simulink model "quad_closed_loop"  (R2024a)
settings: Solver=ode4  StartTime=0.0  StopTime=14  FixedStep=1e-3  RelTol=1e-3
settings Model: Creator=qixiaoyang  LastModifiedBy=qixiaoyang

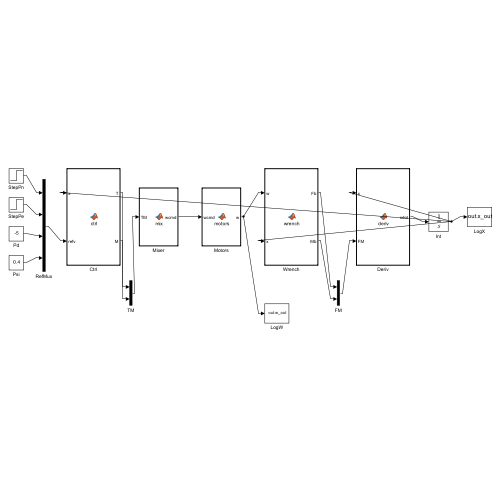
[thumbnail: Simulink's stored preview of the top-level diagram]
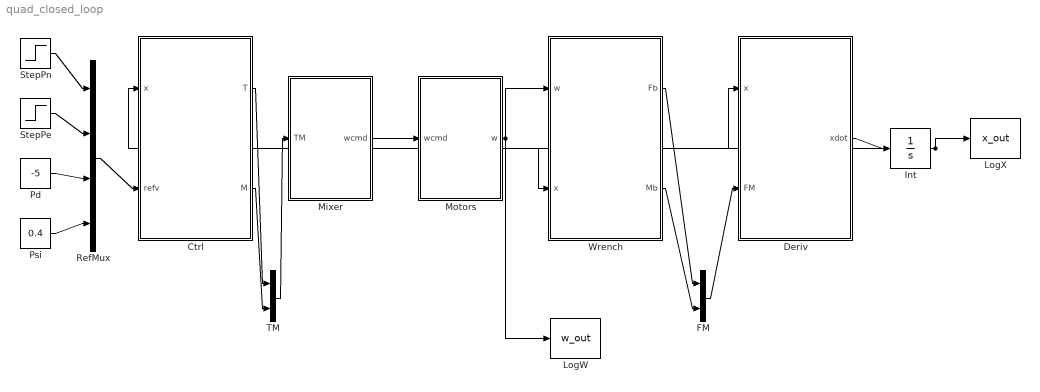
== system quad_closed_loop ==
  Ctrl : MATLAB Function  TreatAsAtomicUnit=on
  Deriv : MATLAB Function  TreatAsAtomicUnit=on
  FM : Mux  Inputs=2
  Int : Integrator  InitialCondition=[0;0;-5;0;0;0;1;0;0;0;0;0;0]
  LogW : ToWorkspace  VariableName=w_out  SaveFormat=Timeseries  SampleTime=-1
  LogX : ToWorkspace  VariableName=x_out  SaveFormat=Timeseries  SampleTime=-1
  Mixer : MATLAB Function  TreatAsAtomicUnit=on
  Motors : MATLAB Function  TreatAsAtomicUnit=on
  Pd : Constant  Value=-5
  Psi : Constant  Value=0.4
  RefMux : Mux
  StepPe : Step  After=2  SampleTime=0
  StepPn : Step  After=3  SampleTime=0
  TM : Mux  Inputs=2
  Wrench : MATLAB Function  TreatAsAtomicUnit=on
  wires:
  StepPn/1 -> RefMux/1
  StepPe/1 -> RefMux/2
  Pd/1 -> RefMux/3
  Psi/1 -> RefMux/4
  Int/1 -> Ctrl/1(x), Wrench/2(x), Deriv/1(x), LogX/1
  RefMux/1 -> Ctrl/2(refv)
  Ctrl/1(T) -> TM/1
  Ctrl/2(M) -> TM/2
  TM/1 -> Mixer/1(TM)
  Mixer/1(wcmd) -> Motors/1(wcmd)
  Motors/1(w) -> Wrench/1(w), LogW/1
  Wrench/1(Fb) -> FM/1
  Wrench/2(Mb) -> FM/2
  FM/1 -> Deriv/2(FM)
  Deriv/1(xdot) -> Int/1

== matlab function quad_closed_loop/Ctrl ==
  settings: updateMethod=DISCRETE  sampleTime=1e-3
  data: x input; T output; refv input; M output
function [T, M] = ctrl(x, refv)
% 级联控制器：位置环 -> 推力方向 -> 姿态环
persistent st
if isempty(st)
    st.ip = [0;0;0];
    st.ia = [0;0;0];
end
pn = x(1:3); Vb = x(4:6); q = x(7:10); w = x(11:13);
R = dcm(q);
Vn = R*Vb;
ep = refv(1:3) - pn;
ev = -Vn;
a = [1.6000000000000001;1.6000000000000001;2.5].*ep + [2.2000000000000002;2.2000000000000002;3].*ev + [0;0;1.2].*st.ip;
aHor = a(1:2);
aMax = 9.8100000000000005*tan(0.6108652381980153);
if norm(aHor) > aMax
    a(1:2) = aHor*(aMax/norm(aHor));
end
st.ip = st.ip + ep*0.001;
st.ip = min(max(st.ip, -[0;0;1]), [0;0;1]);
v = [0;0;9.8100000000000005] - a;
nv = norm(v);
if nv < 1e-6
    v = [0;0;1]; nv = 1;
end
z = v/nv;
T = 1.5*nv;
T = min(max(T, 0), 40);
psi = refv(4);
xc = [cos(psi); sin(psi); 0];
yb = cross(z, xc);
ny = norm(yb);
if ny < 1e-6
    xc = [1;0;0]; yb = cross(z, xc); ny = norm(yb);
end
yb = yb/ny;
xb = cross(yb, z);
Rd = [xb yb z];
phiD = atan2(Rd(3,2), Rd(3,3));
thetaD = -asin(max(-1, min(1, Rd(3,1))));
psiD = atan2(Rd(2,1), Rd(1,1));
att = euler(q);
e = [phiD;thetaD;psiD] - att;
e = mod(e + pi, 2*pi) - pi;
st.ia = st.ia + e*0.001;
st.ia = min(max(st.ia, -[0.20000000000000001;0.20000000000000001;0.20000000000000001]), [0.20000000000000001;0.20000000000000001;0.20000000000000001]);
M = [6;6;3].*e + [0;0;0.14999999999999999].*st.ia - [0.34999999999999998;0.34999999999999998;0.29999999999999999].*w;
M = min(max(M, -[3;3;1.5]), [3;3;1.5]);
end
function R = dcm(q)
n = norm(q);
if n < 1e-12, q = [1;0;0;0]; else, q = q/n; end
w = q(1); x = q(2); y = q(3); z = q(4);
R = [1-2*(y*y+z*z), 2*(x*y-w*z), 2*(x*z+w*y);
     2*(x*y+w*z), 1-2*(x*x+z*z), 2*(y*z-w*x);
     2*(x*z-w*y), 2*(y*z+w*x), 1-2*(x*x+y*y)];
end
function e = euler(q)
n = norm(q);
if n < 1e-12, e = [0;0;0]; return; end
q = q/n;
w = q(1); x = q(2); y = q(3); z = q(4);
s2 = 2*(w*y - z*x);
s2 = max(-1, min(1, s2));
e = [atan2(2*(w*x + y*z), 1 - 2*(x*x + y*y));
     asin(s2);
     atan2(2*(w*z + x*y), 1 - 2*(y*y + z*z))];
end

== matlab function quad_closed_loop/Motors ==
  settings: updateMethod=DISCRETE  sampleTime=1e-3
  data: wcmd input; w output
function w = motors(wcmd)
% 一阶电机模型，按 1 ms 步长解析离散
persistent w0
if isempty(w0), w0 = 495.22722057657535*ones(4,1); end
alpha = exp(-0.001/0.02);
w0 = wcmd + (w0 - wcmd)*alpha;
w0 = min(max(w0, 0), 1200);
w = w0;
end

== matlab function quad_closed_loop/Wrench ==
  data: w input; Fb output; x input; Mb output
function [Fb, Mb] = wrench(w, x)
% 旋翼推力与反扭矩，含机体轴线性阻力
Vb = x(4:6);
Tid = 1.5e-05 * w.^2;
Fb = [0;0;-sum(Tid)] - 0.080000000000000002*Vb;
Mb = [-0.15909902576697318*(Tid(1) + Tid(2)) + 0.15909902576697318*(Tid(3) + Tid(4));
       0.15909902576697318*(Tid(1) - Tid(2) - Tid(3) + Tid(4));
       0.013333333333333332*(Tid(1) - Tid(2) + Tid(3) - Tid(4))];
end

== matlab function quad_closed_loop/Deriv ==
  data: x input; xdot output; FM input
function xdot = deriv(x, FM)
% 刚体六自由度：世界 NED，机体 FRD，状态 13 维
Fb = FM(1:3); Mb = FM(4:6);
Vb = x(4:6); q = x(7:10); w = x(11:13);
R = dcm(q);
qd = 0.5*qmul(q, [0;w]);
Vbd = Fb/1.5 - cross(w, Vb) + R'*[0;0;9.8100000000000005];
I = [0.0035000000000000001 0 0; 0 0.0035000000000000001 0; 0 0 0.0064999999999999997];
wd = I \ (Mb - cross(w, I*w));
xdot = [R*Vb; Vbd; qd; wd];
end
function R = dcm(q)
n = norm(q);
if n < 1e-12, q = [1;0;0;0]; else, q = q/n; end
w = q(1); x = q(2); y = q(3); z = q(4);
R = [1-2*(y*y+z*z), 2*(x*y-w*z), 2*(x*z+w*y);
     2*(x*y+w*z), 1-2*(x*x+z*z), 2*(y*z-w*x);
     2*(x*z-w*y), 2*(y*z+w*x), 1-2*(x*x+y*y)];
end
function r = qmul(a, b)
aw = a(1); av = a(2:4);
bw = b(1); bv = b(2:4);
r = [aw*bw - av'*bv; aw*bv + bw*av + cross(av, bv)];
end

== matlab function quad_closed_loop/Mixer ==
  data: TM input; wcmd output
function wcmd = mix(TM)
% 混控：力/力矩 -> 转速，负的转速平方截断为 0
w2 = [16666.666666666679 -104756.56017578482 104756.56017578482 1250000;16666.666666666664 -104756.56017578482 -104756.56017578482 -1250000;16666.666666666664 104756.56017578482 -104756.56017578482 1250000;16666.666666666664 104756.56017578482 104756.56017578482 -1250000] * TM;
w2 = max(w2, 0);
wcmd = sqrt(w2);
wcmd = min(wcmd, 1200);
end
